simulink model "fixYawControl"  (R2026b)
settings: Solver=VariableStepAuto  StopTime=100
model workspace (MAT data in the model file):
  g = 9.81
  m = 5.43122
undefined symbols (not defined in the file or in its folder): X, Y, Z
libraries: sm_lib x15, nesl_utility x8, sdl_lib x4, slpidlib x4
(part 2 of 2)

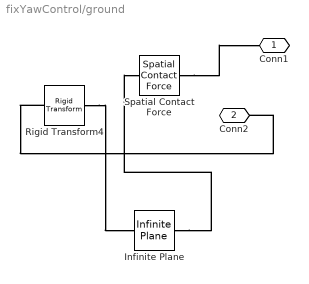
== system fixYawControl/ground ==
  Infinite Plane : sm_lib/Curves and Surfaces/Infinite Plane  GraphicType=Rectangle  GraphicPlaneWidth=1  GraphicPlaneWidthUnits=m  GraphicPlaneHeight=1  GraphicPlaneHeightUnits=m  GraphicVisPropType=SimpleVisualProperties  GraphicDiffuseColor=[0.5 0.5 0.5]  GraphicOpacity=1  GraphicSpecularColor=[0.5 0.5 0.5 1.0]  GraphicAmbientColor=[0.15 0.15 0.15 1.0]  GraphicEmissiveColor=[0.0 0.0 0.0 1.0]  GraphicShininess=75
  Rigid Transform4 : sm_lib/Frames and Transforms/Rigid Transform  RotationMethod=None  FollAlignAxisA=+X  BaseAlignAxisA=+Y  FollAlignAxisB=+Y  BaseAlignAxisB=+Z  RotationStandardAxis=+Z  RotationAngle=0  RotationAngleUnits=deg  RotationArbitraryAxis=[0 0 1]  RotationSequenceAxes=FollowerAxes  RotationSequence=XYX  RotationSequenceAngles=[0 0 0]  RotationSequenceAnglesUnits=deg  RotationMatrix=[1 0 0;0 1 0;0 0 1]  Quaternion=[1 0 0 0]  TranslationMethod=Cartesian  TranslationCartesianOffset=[0 0 -0.3]  TranslationCartesianOffsetUnits=m  TranslationStandardAxis=+Z  TranslationStandardOffset=0  TranslationStandardOffsetUnits=m  TranslationROffset=0  TranslationROffsetUnits=m  TranslationThetaOffset=0  TranslationThetaOffsetUnits=deg  TranslationZOffset=0  TranslationZOffsetUnits=m
  Spatial Contact Force : sm_lib/Forces and Torques/Spatial Contact Force  SenseSeparationDistance=off  NormalForceType=SmoothSpringDamper  NormalStiffness=1e6  NormalStiffnessUnits=N/m  NormalDamping=1e3  NormalDampingUnits=N/(m/s)  NormalTransitionRegionWidth=1e-4  NormalTransitionRegionWidthUnits=m  FrictionType=SmoothStickSlip  CoefficientOfStaticFriction=0.5  CoefficientOfDynamicFriction=0.3  FrictionalCriticalVelocity=1e-3  FrictionalCriticalVelocityUnits=m/s  SenseContactSignal=off  SensePenetrationDepth=off  SenseNormalVelocity=off  SenseTangentialVelocity=off  SensingForceTorqueDirection=BaseOnFollower  SensingForceTorqueResolutionFrame=ContactFrame  SenseNormalForce=off  SenseNormalForceMagnitude=off  SenseNormalTorque=off  SenseFrictionalForce=off  SenseFrictionalForceMagnitude=off  SenseFrictionalTorque=off  SenseTotalForce=off  SenseTotalTorque=off  SenseContactBaseRotation=off  SenseContactBaseTranslation=off  SenseContactFollowerRotation=off  SenseContactFollowerTranslation=off  ZeroCrossDetectContactStartAndEnd=off
  Conn1 : PMIOPort  Side=Left
  Conn2 : PMIOPort  Port=2  Side=Right
  connections:
  Infinite Plane/RConn1 -- Spatial Contact Force/LConn1
  Rigid Transform4/RConn1 -- Infinite Plane/LConn1
  Spatial Contact Force/RConn1 -- Conn1/RConn1
  Rigid Transform4/LConn1 -- Conn2/RConn1

== matlab function fixYawControl/MATLAB Function1 ==
  data: rpm_col input; rpm_M1 output; u_roll input; u_pitch input; rpm_M2 output; rpm_M3 output; rpm_M4 output; u_yaw input

function [rpm_M1, rpm_M2, rpm_M3, rpm_M4] = MotorMixer(rpm_col, u_roll, u_pitch, u_yaw)
%#codegen

rpm_M1 = rpm_col + u_roll + u_pitch - u_yaw;
rpm_M2 = rpm_col - u_roll + u_pitch + u_yaw;
rpm_M3 = rpm_col + u_roll - u_pitch + u_yaw;
rpm_M4 = rpm_col - u_roll - u_pitch - u_yaw;

end

== matlab function fixYawControl/MATLAB Function ==
  data: Q input; rotX output; rotY output; rotZ output
function [rotX, rotY, rotZ] = quatToEuler(Q)
% Q = [q0 q1 q2 q3], scalar first

q0 = Q(1);
q1 = Q(2);
q2 = Q(3);
q3 = Q(4);

rotX = atan2(2*(q0*q1 + q2*q3), ...
    1 - 2*(q1^2 + q2^2));

s = 2*(q0*q2 - q3*q1);
s = max(-1, min(1, s));
rotY = asin(s);

rotZ = atan2(2*(q0*q3 + q1*q2), ...
    1 - 2*(q2^2 + q3^2));
end
